simulink model "hopper_6dof"  (R2026b)
settings: Solver=FixedStepAuto  StopTime=tgrid(end)  FixedStep=1e-3  RelTol=1e-5
undefined symbols (not defined in the file): cg_init, controller_start_time, fdir_params, fsw_latency, fsw_period, g, IN, K1flat, K1flat_lo, K2grid, Klqi, nav_dt, nav_g, nav_init, nav_Qc, nav_reset, OUT, p, sensor_params, Target_Trajectory, tgrid, u_hold_command, unom, VEH
libraries: fl_lib x43, nesl_utility x31, SimscapeFluids_lib x13, slpidlib x3, simulink_extras x2, commrandsrc3 x1, dspsrcs4 x1, matrix_library x1, aerolibutil x1
(part 2 of 6)

== system hopper_6dof/Logging/Scopes_slosh/On ==
  dyn_bus : Inport
  mux : Mux  Inputs=2
  sel_dyn_bus : BusSelector  OutputSignals=ox_slosh_pos,fu_slosh_pos,ox_slosh_mass,fu_slosh_mass,f_body,cg_accel
  slosh : Scope  NumInputPorts=5
      settings: ActiveDisplayString=5  Title=CG acceleration (m/s^2)
  wires:
  mux/1 -> slosh/3
  sel_dyn_bus/5 -> slosh/4  "<f_body>"
  sel_dyn_bus/3 -> mux/1  "<ox_slosh_mass>"
  sel_dyn_bus/1 -> slosh/1  "<ox_slosh_pos>"
  dyn_bus/1 -> sel_dyn_bus/1
  sel_dyn_bus/6 -> slosh/5  "<cg_accel>"
  sel_dyn_bus/4 -> mux/2  "<fu_slosh_mass>"
  sel_dyn_bus/2 -> slosh/2  "<fu_slosh_pos>"

== system hopper_6dof/Logging/Scopes_trajectory/On ==
  dyn_bus : Inport
  mux : Mux  Inputs=2
  mux1 : Mux  Inputs=2
  mux2 : Mux  Inputs=2
  sel_dyn_bus : BusSelector  OutputSignals=x,y,z,w,vel_ned
  trajectory : Scope  NumInputPorts=4
      settings: ActiveDisplayString=4  Title=Velocity NED (m/s)  ActiveDisplayYMinimum=-1.7884841658512411  ActiveDisplayYMaximum=1.6649835435575939
  vz_ref_ts : FromWorkspace  VariableName=vz_ref_ts
  z_ref_ts : FromWorkspace  VariableName=z_ref_ts
  wires:
  sel_dyn_bus/5 -> trajectory/4  "<vel_ned>"
  sel_dyn_bus/3 -> mux1/1  "<z>"
  sel_dyn_bus/1 -> mux/1  "<x>"
  dyn_bus/1 -> sel_dyn_bus/1
  sel_dyn_bus/4 -> mux2/1  "<w>"
  sel_dyn_bus/2 -> mux/2  "<y>"
  z_ref_ts/1 -> mux1/2  "z_ref_ts"
  vz_ref_ts/1 -> mux2/2  "vz_ref_ts"
  mux/1 -> trajectory/1
  mux1/1 -> trajectory/2
  mux2/1 -> trajectory/3

== system hopper_6dof/Logging/Signal_Dump/On ==
  env_bus : Inport
  nav_bus : Inport  Port=2
  gnc_bus : Inport  Port=3
  act_bus : Inport  Port=4
  prop_bus : Inport  Port=5
  dyn_bus : Inport  Port=6
  end_act_bus : Terminator
  end_dyn_bus : Terminator
  end_env_bus : Terminator
  end_gnc_bus : Terminator
  end_nav_bus : Terminator
  end_prop_bus : Terminator
  wires:
  env_bus/1 -> end_env_bus/1
  nav_bus/1 -> end_nav_bus/1
  gnc_bus/1 -> end_gnc_bus/1
  act_bus/1 -> end_act_bus/1
  prop_bus/1 -> end_prop_bus/1
  dyn_bus/1 -> end_dyn_bus/1

== system hopper_6dof/Mass_Propulsion/Propellant_Flow/Flow_Constant ==
  Ox_mdot_in : Inport
  Fu_mdot_in : Inport  Port=2
  Unused1 : Terminator
  Unused2 : Terminator
  Zero1 : Constant  Value=0
  Zero2 : Constant  Value=0
  Ox_mdot : Outport
  Fu_mdot : Outport  Port=2
  wires:
  Ox_mdot_in/1 -> Unused1/1
  Fu_mdot_in/1 -> Unused2/1
  Zero1/1 -> Ox_mdot/1
  Zero2/1 -> Fu_mdot/1

== system hopper_6dof/Mass_Propulsion/Propellant_Flow/Flow_Varying ==
  Ox_mdot_in : Inport
  Fu_mdot_in : Inport  Port=2
  Ox_mdot : Outport
  Fu_mdot : Outport  Port=2
  wires:
  Ox_mdot_in/1 -> Ox_mdot/1
  Fu_mdot_in/1 -> Fu_mdot/1

== system hopper_6dof/Mass_Propulsion/Propulsion/Propulsion_Fluid_Network ==
  Thrust_Cmd : Inport
  Fluid_Network : Subsystem
  Thrust : Outport
  Ox_mdot : Outport  Port=2
  Fu_mdot : Outport  Port=3
  wires:
  Thrust_Cmd/1 -> Fluid_Network/1(F_cmd)
  Fluid_Network/1(Actual Thrust) -> Thrust/1  "actual_thrust_N"
  Fluid_Network/2(Actual Ox mdot) -> Ox_mdot/1  "actual_ox_mdot_kgps"
  Fluid_Network/3(Actual Fuel mdot) -> Fu_mdot/1  "actual_fuel_mdot_kgps"

== system hopper_6dof/Mass_Propulsion/Propulsion/Propulsion_LUT ==
  Thrust_Cmd : Inport
  Thrust_to_Mdot_LUT : Subsystem  ReferencedSubsystem=Thrust_to_Mdot_LUT
  Thrust : Outport
  Ox_mdot : Outport  Port=2
  Fu_mdot : Outport  Port=3
  wires:
  Thrust_Cmd/1 -> Thrust/1, Thrust_to_Mdot_LUT/1
  Thrust_to_Mdot_LUT/1 -> Ox_mdot/1
  Thrust_to_Mdot_LUT/2 -> Fu_mdot/1

== system hopper_6dof/Navigation_Sensors/FSW_Sensor_Ports/FSW_Sensor_Ports_On ==
  meas : Inport
  valid : Inport  Port=2
  stamp : Inport  Port=3
  sens_meas : Outport
  sens_valid : Outport  Port=2
  sens_stamp : Outport  Port=3
  wires:
  meas/1 -> sens_meas/1
  valid/1 -> sens_valid/1
  stamp/1 -> sens_stamp/1

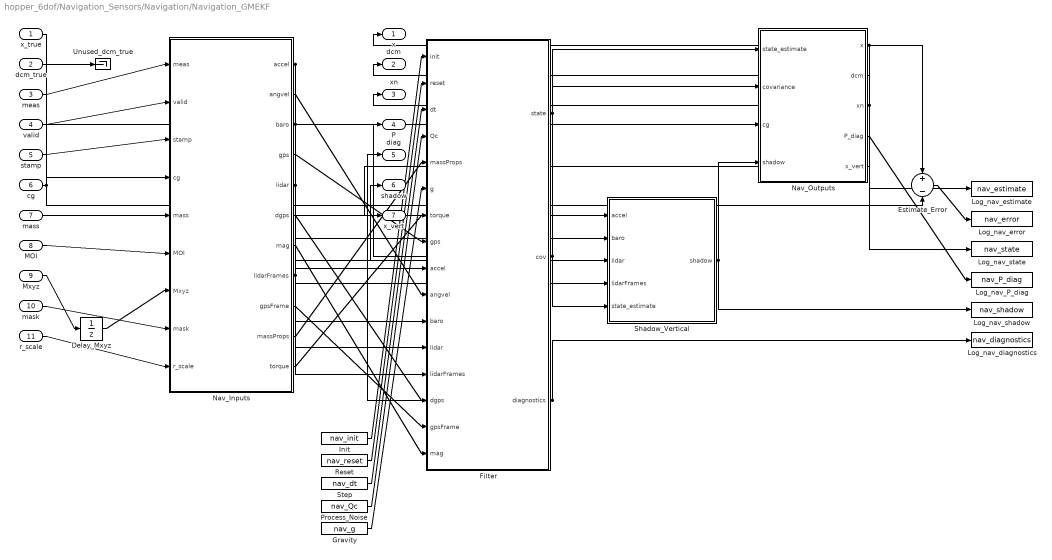
== system hopper_6dof/Navigation_Sensors/Navigation/Navigation_GMEKF ==
  x_true : Inport
  dcm_true : Inport  Port=2
  meas : Inport  Port=3
  valid : Inport  Port=4
  stamp : Inport  Port=5
  cg : Inport  Port=6
  mass : Inport  Port=7
  MOI : Inport  Port=8
  Mxyz : Inport  Port=9
  mask : Inport  Port=10
  r_scale : Inport  Port=11
  Delay_Mxyz : UnitDelay  InitialCondition=zeros(3,1)  SampleTime=nav_dt
  Estimate_Error : Sum  Inputs=+-
  Filter : Subsystem  Variant=on
  Gravity : Constant  Value=nav_g
  Init : Constant  Value=nav_init  OutDataTypeStr=Bus: InitConditions
  Log_nav_P_diag : ToWorkspace  VariableName=nav_P_diag  SaveFormat=Timeseries
  Log_nav_diagnostics : ToWorkspace  VariableName=nav_diagnostics  SaveFormat=Timeseries
  Log_nav_error : ToWorkspace  VariableName=nav_error  SaveFormat=Timeseries
  Log_nav_estimate : ToWorkspace  VariableName=nav_estimate  SaveFormat=Timeseries
  Log_nav_shadow : ToWorkspace  VariableName=nav_shadow  SaveFormat=Timeseries
  Log_nav_state : ToWorkspace  VariableName=nav_state  SaveFormat=Timeseries
  Nav_Inputs : MATLAB Function  TreatAsAtomicUnit=on  SystemSampleTime=nav_dt
  Nav_Outputs : MATLAB Function  TreatAsAtomicUnit=on
  Process_Noise : Constant  Value=nav_Qc
  Reset : Constant  Value=nav_reset
  Shadow_Vertical : MATLAB Function  TreatAsAtomicUnit=on  SystemSampleTime=nav_dt
  Step : Constant  Value=nav_dt
  Unused_dcm_true : Terminator
  x : Outport
  dcm : Outport  Port=2
  xn : Outport  Port=3
  P : Outport  Port=4
  diag : Outport  Port=5
  shadow : Outport  Port=6
  x_vert : Outport  Port=7
  wires:
  Mxyz/1 -> Delay_Mxyz/1
  meas/1 -> Nav_Inputs/1(meas)
  valid/1 -> Nav_Inputs/2(valid)
  stamp/1 -> Nav_Inputs/3(stamp)
  cg/1 -> Nav_Inputs/4(cg), Nav_Outputs/3(cg)
  mass/1 -> Nav_Inputs/5(mass)
  MOI/1 -> Nav_Inputs/6(MOI)
  Delay_Mxyz/1 -> Nav_Inputs/7(Mxyz)
  mask/1 -> Nav_Inputs/8(mask)
  r_scale/1 -> Nav_Inputs/9(r_scale)
  Init/1 -> Filter/1(init)
  Reset/1 -> Filter/2(reset)
  Step/1 -> Filter/3(dt)
  Process_Noise/1 -> Filter/4(Qc)
  Nav_Inputs/10(massProps) -> Filter/5(massProps)
  Gravity/1 -> Filter/6(g)
  Nav_Inputs/11(torque) -> Filter/7(torque)
  Nav_Inputs/4(gps) -> Filter/8(gps)
  Nav_Inputs/1(accel) -> Filter/9(accel), Shadow_Vertical/1(accel)
  Nav_Inputs/2(angvel) -> Filter/10(angvel)
  Nav_Inputs/3(baro) -> Filter/11(baro), Shadow_Vertical/2(baro)
  Nav_Inputs/5(lidar) -> Filter/12(lidar), Shadow_Vertical/3(lidar)
  Nav_Inputs/8(lidarFrames) -> Filter/13(lidarFrames), Shadow_Vertical/4(lidarFrames)
  Nav_Inputs/6(dgps) -> Filter/14(dgps)
  Nav_Inputs/9(gpsFrame) -> Filter/15(gpsFrame)
  Nav_Inputs/7(mag) -> Filter/16(mag)
  Filter/1(state) -> Shadow_Vertical/5(state_estimate), Nav_Outputs/1(state_estimate)
  Filter/2(cov) -> Nav_Outputs/2(covariance), P/1
  Shadow_Vertical/1(shadow) -> Nav_Outputs/4(shadow), shadow/1, Log_nav_shadow/1
  Nav_Outputs/3(xn) -> xn/1, Log_nav_state/1
  Filter/3(diagnostics) -> diag/1, Log_nav_diagnostics/1
  Nav_Outputs/1(x) -> Estimate_Error/1, Log_nav_estimate/1, x/1
  x_true/1 -> Estimate_Error/2
  Estimate_Error/1 -> Log_nav_error/1
  Nav_Outputs/4(P_diag) -> Log_nav_P_diag/1
  Nav_Outputs/2(dcm) -> dcm/1
  Nav_Outputs/5(x_vert) -> x_vert/1
  dcm_true/1 -> Unused_dcm_true/1

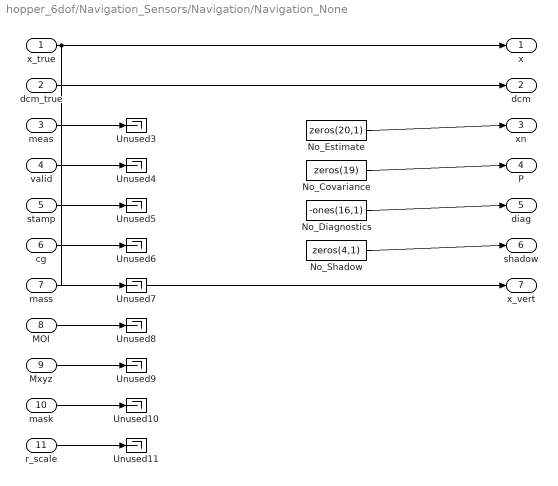
== system hopper_6dof/Navigation_Sensors/Navigation/Navigation_None ==
  x_true : Inport
  dcm_true : Inport  Port=2
  meas : Inport  Port=3
  valid : Inport  Port=4
  stamp : Inport  Port=5
  cg : Inport  Port=6
  mass : Inport  Port=7
  MOI : Inport  Port=8
  Mxyz : Inport  Port=9
  mask : Inport  Port=10
  r_scale : Inport  Port=11
  No_Covariance : Constant  Value=zeros(19)
  No_Diagnostics : Constant  Value=-ones(16,1)
  No_Estimate : Constant  Value=zeros(20,1)
  No_Shadow : Constant  Value=zeros(4,1)
  Unused{3..11} (9 alike) : Terminator
  x : Outport
  dcm : Outport  Port=2
  xn : Outport  Port=3
  P : Outport  Port=4
  diag : Outport  Port=5
  shadow : Outport  Port=6
  x_vert : Outport  Port=7
  wires:
  x_true/1 -> x/1, x_vert/1
  dcm_true/1 -> dcm/1
  No_Estimate/1 -> xn/1
  No_Covariance/1 -> P/1
  No_Diagnostics/1 -> diag/1
  No_Shadow/1 -> shadow/1
  meas/1 -> Unused3/1
  valid/1 -> Unused4/1
  stamp/1 -> Unused5/1
  cg/1 -> Unused6/1
  mass/1 -> Unused7/1
  MOI/1 -> Unused8/1
  Mxyz/1 -> Unused9/1
  mask/1 -> Unused10/1
  r_scale/1 -> Unused11/1

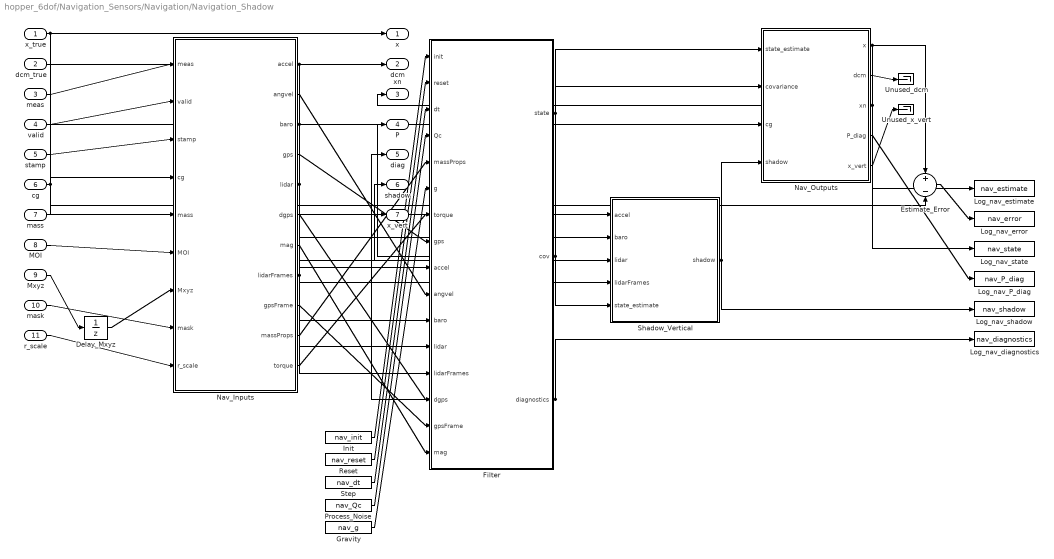
== system hopper_6dof/Navigation_Sensors/Navigation/Navigation_Shadow ==
  x_true : Inport
  dcm_true : Inport  Port=2
  meas : Inport  Port=3
  valid : Inport  Port=4
  stamp : Inport  Port=5
  cg : Inport  Port=6
  mass : Inport  Port=7
  MOI : Inport  Port=8
  Mxyz : Inport  Port=9
  mask : Inport  Port=10
  r_scale : Inport  Port=11
  Delay_Mxyz : UnitDelay  InitialCondition=zeros(3,1)  SampleTime=nav_dt
  Estimate_Error : Sum  Inputs=+-
  Filter : Subsystem  Variant=on
  Gravity : Constant  Value=nav_g
  Init : Constant  Value=nav_init  OutDataTypeStr=Bus: InitConditions
  Log_nav_P_diag : ToWorkspace  VariableName=nav_P_diag  SaveFormat=Timeseries
  Log_nav_diagnostics : ToWorkspace  VariableName=nav_diagnostics  SaveFormat=Timeseries
  Log_nav_error : ToWorkspace  VariableName=nav_error  SaveFormat=Timeseries
  Log_nav_estimate : ToWorkspace  VariableName=nav_estimate  SaveFormat=Timeseries
  Log_nav_shadow : ToWorkspace  VariableName=nav_shadow  SaveFormat=Timeseries
  Log_nav_state : ToWorkspace  VariableName=nav_state  SaveFormat=Timeseries
  Nav_Inputs : MATLAB Function  TreatAsAtomicUnit=on  SystemSampleTime=nav_dt
  Nav_Outputs : MATLAB Function  TreatAsAtomicUnit=on
  Process_Noise : Constant  Value=nav_Qc
  Reset : Constant  Value=nav_reset
  Shadow_Vertical : MATLAB Function  TreatAsAtomicUnit=on  SystemSampleTime=nav_dt
  Step : Constant  Value=nav_dt
  Unused_dcm : Terminator
  Unused_x_vert : Terminator
  x : Outport
  dcm : Outport  Port=2
  xn : Outport  Port=3
  P : Outport  Port=4
  diag : Outport  Port=5
  shadow : Outport  Port=6
  x_vert : Outport  Port=7
  wires:
  Mxyz/1 -> Delay_Mxyz/1
  meas/1 -> Nav_Inputs/1(meas)
  valid/1 -> Nav_Inputs/2(valid)
  stamp/1 -> Nav_Inputs/3(stamp)
  cg/1 -> Nav_Inputs/4(cg), Nav_Outputs/3(cg)
  mass/1 -> Nav_Inputs/5(mass)
  MOI/1 -> Nav_Inputs/6(MOI)
  Delay_Mxyz/1 -> Nav_Inputs/7(Mxyz)
  mask/1 -> Nav_Inputs/8(mask)
  r_scale/1 -> Nav_Inputs/9(r_scale)
  Init/1 -> Filter/1(init)
  Reset/1 -> Filter/2(reset)
  Step/1 -> Filter/3(dt)
  Process_Noise/1 -> Filter/4(Qc)
  Nav_Inputs/10(massProps) -> Filter/5(massProps)
  Gravity/1 -> Filter/6(g)
  Nav_Inputs/11(torque) -> Filter/7(torque)
  Nav_Inputs/4(gps) -> Filter/8(gps)
  Nav_Inputs/1(accel) -> Filter/9(accel), Shadow_Vertical/1(accel)
  Nav_Inputs/2(angvel) -> Filter/10(angvel)
  Nav_Inputs/3(baro) -> Filter/11(baro), Shadow_Vertical/2(baro)
  Nav_Inputs/5(lidar) -> Filter/12(lidar), Shadow_Vertical/3(lidar)
  Nav_Inputs/8(lidarFrames) -> Filter/13(lidarFrames), Shadow_Vertical/4(lidarFrames)
  Nav_Inputs/6(dgps) -> Filter/14(dgps)
  Nav_Inputs/9(gpsFrame) -> Filter/15(gpsFrame)
  Nav_Inputs/7(mag) -> Filter/16(mag)
  Filter/1(state) -> Shadow_Vertical/5(state_estimate), Nav_Outputs/1(state_estimate)
  Filter/2(cov) -> Nav_Outputs/2(covariance), P/1
  Shadow_Vertical/1(shadow) -> Nav_Outputs/4(shadow), shadow/1, Log_nav_shadow/1
  Nav_Outputs/3(xn) -> xn/1, Log_nav_state/1
  Filter/3(diagnostics) -> diag/1, Log_nav_diagnostics/1
  Nav_Outputs/1(x) -> Estimate_Error/1, Log_nav_estimate/1
  x_true/1 -> Estimate_Error/2, x/1, x_vert/1
  Estimate_Error/1 -> Log_nav_error/1
  Nav_Outputs/4(P_diag) -> Log_nav_P_diag/1
  dcm_true/1 -> dcm/1
  Nav_Outputs/2(dcm) -> Unused_dcm/1
  Nav_Outputs/5(x_vert) -> Unused_x_vert/1

== system hopper_6dof/Navigation_Sensors/Sensors/Sensors_Off ==
  x : Inport
  f_b : Inport  Port=2
  dcm_be : Inport  Port=3
  cg : Inport  Port=4
  Unused{1..4} (4 alike) : Terminator
  Zero1 : Constant  Value=zeros(26,1)
  Zero2 : Constant  Value=zeros(9,1)
  Zero3 : Constant  Value=zeros(9,1)
  meas : Outport
  valid : Outport  Port=2
  stamp : Outport  Port=3
  wires:
  x/1 -> Unused1/1
  f_b/1 -> Unused2/1
  dcm_be/1 -> Unused3/1
  cg/1 -> Unused4/1
  Zero1/1 -> meas/1
  Zero2/1 -> valid/1
  Zero3/1 -> stamp/1

== system hopper_6dof/Navigation_Sensors/Sensors/Sensors_On ==
  x : Inport
  f_b : Inport  Port=2
  dcm_be : Inport  Port=3
  cg : Inport  Port=4
  Clock : Clock
  Sensor_Frame : MATLAB Function  TreatAsAtomicUnit=on  SystemSampleTime=sensor_params.dt
  Sensor_Noise : RandomNumber  Mean=zeros(26,1)  Variance=ones(26,1)  Seed=sensor_params.S.seed + (0:25)'  SampleTime=sensor_params.dt
  meas : Outport
  valid : Outport  Port=2
  stamp : Outport  Port=3
  wires:
  Clock/1 -> Sensor_Frame/1(t)
  Sensor_Noise/1 -> Sensor_Frame/2(noise)
  x/1 -> Sensor_Frame/3(x)
  f_b/1 -> Sensor_Frame/4(f_b)
  dcm_be/1 -> Sensor_Frame/5(dcm_be)
  cg/1 -> Sensor_Frame/6(cg)
  Sensor_Frame/1(meas) -> meas/1
  Sensor_Frame/2(valid) -> valid/1
  Sensor_Frame/3(stamp) -> stamp/1

== system hopper_6dof/Vehicle_Dynamics/Ground_Contact/Ground_None ==
  Inertial Position : Inport
  Inertial Velocity : Inport  Port=2
  Inertial to Body : Inport  Port=3
  Angular Velocity : Inport  Port=4
  Unused{1..4} (4 alike) : Terminator
  Zero1 : Constant  Value=[0 0 0]
  Zero2 : Constant  Value=[0 0 0]
  Body Force : Outport
  Body Moment : Outport  Port=2
  wires:
  Inertial Position/1 -> Unused1/1
  Inertial Velocity/1 -> Unused2/1
  Inertial to Body/1 -> Unused3/1
  Angular Velocity/1 -> Unused4/1
  Zero1/1 -> Body Force/1
  Zero2/1 -> Body Moment/1

== system hopper_6dof/Vehicle_Dynamics/Ground_Contact/Ground_Strut ==
  Inertial Position : Inport
  Inertial Velocity : Inport  Port=2
  Inertial to Body : Inport  Port=3
  Angular Velocity : Inport  Port=4
  Ground_Contact : Subsystem  ReferencedSubsystem=Ground_Contact
  Body Force : Outport
  Body Moment : Outport  Port=2
  wires:
  Inertial Position/1 -> Ground_Contact/1
  Inertial Velocity/1 -> Ground_Contact/2
  Inertial to Body/1 -> Ground_Contact/3
  Angular Velocity/1 -> Ground_Contact/4
  Ground_Contact/1 -> Body Force/1
  Ground_Contact/2 -> Body Moment/1

== system hopper_6dof/Vehicle_Dynamics/Slosh/Slosh_Off ==
  Ox mass : Inport
  Fuel mass : Inport  Port=2
  CG Acceleration : Inport  Port=3
  Angular Velocity : Inport  Port=4
  Angular Acceleration : Inport  Port=5
  CG Location : Inport  Port=6
  Unused{1..6} (6 alike) : Terminator
  Zero{1,3..6} (5 alike) : Constant  Value=[0 0 0]
  Zero2 : Constant  Value=zeros(3,1)
  Slosh_F : Outport
  Slosh_M : Outport  Port=2
  ox_slosh_pos : Outport  Port=3
  ox_slosh_mass : Outport  Port=4
  fu_slosh_pos : Outport  Port=5
  fu_slosh_mass : Outport  Port=6
  wires:
  Ox mass/1 -> Unused1/1
  Fuel mass/1 -> Unused2/1
  CG Acceleration/1 -> Unused3/1
  Angular Velocity/1 -> Unused4/1
  Angular Acceleration/1 -> Unused5/1
  CG Location/1 -> Unused6/1
  Zero1/1 -> Slosh_F/1
  Zero2/1 -> Slosh_M/1
  Zero3/1 -> ox_slosh_pos/1
  Zero4/1 -> ox_slosh_mass/1
  Zero5/1 -> fu_slosh_pos/1
  Zero6/1 -> fu_slosh_mass/1

== system hopper_6dof/GNC/Controller/Controller_LQI/MRP Correction ==
  In1 : Inport
  Constant : Constant  Value=p(2)
  Demux : Demux  Outputs=3
  Mux : Mux  Inputs=3
  Sum : Sum  Inputs=|+-
  Out1 : Outport
  wires:
  Demux/1 -> Mux/1
  Demux/3 -> Mux/3
  Constant/1 -> Sum/2
  Mux/1 -> Out1/1
  Sum/1 -> Mux/2
  Demux/2 -> Sum/1
  In1/1 -> Demux/1

== system hopper_6dof/GNC/Controller/Controller_LQI/q to MRP ==
  In1 : Inport
  Constant : Constant
  Matrix Divide : Product  Inputs=*/
  Selector : Selector  InputPortWidth=4  IndexOptions=Index vector (dialog)  Indices=[1 2 3]  OutputSizes=1  RuntimeRangeChecks=off
  Selector1 : Selector  InputPortWidth=4  IndexOptions=Index vector (dialog)  Indices=[1]  OutputSizes=1  RuntimeRangeChecks=off
  Sum : Sum  Inputs=|++
  Out1 : Outport
  wires:
  Matrix Divide/1 -> Out1/1
  Sum/1 -> Matrix Divide/2
  Selector/1 -> Matrix Divide/1
  Constant/1 -> Sum/2
  Selector1/1 -> Sum/1
  In1/1 -> Selector/1, Selector1/1

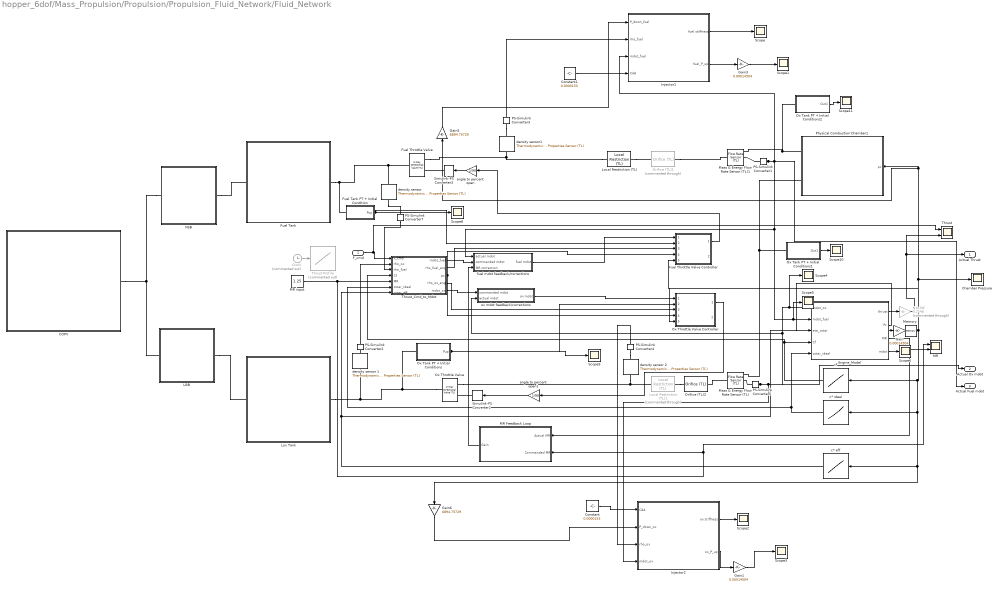
== system hopper_6dof/Mass_Propulsion/Propulsion/Propulsion_Fluid_Network/Fluid_Network ==
  F_cmd : Inport
  COPV : Subsystem
  Chamber Pressure : Scope
      settings: ActiveDisplayYMinimum=24.4768520913143  ActiveDisplayYMaximum=276.14956071215624  DataLoggingVariableName=ScopeData22
  Clock : Clock  Commented=on
  Constant : Constant  Value=0.0000153
  Constant1 : Constant  Value=0.0000153
  Engine_Model : MATLAB Function  TreatAsAtomicUnit=on
  FBB : Subsystem
  Fuel Tank : Subsystem
  Fuel Tank PT + Initial Condition : Subsystem
  Fuel Throttle Valve : SimscapeFluids_lib/Thermal Liquid/Valves & Orifices/Directional Control Valves/2-Way Directional Valve (TL)  valve_spec=fluids.thermal_liquid.valves.directional_control_valves.enum.ValveSpec.Table1DAreaOpening  S_max=1 m  del_S_max=5e-3 m  area_max=1e-4 m^2  area_leak=1e-10 m^2  del_S_TLU=[0 0.3 0.4 0.5 0.6 0.7 0.8 0.9 1.0] m  valve_area_TLU=[1e-9 1.7065e-07 1.0239e-06 3.5836e-06 7.8498e-06 1.4164e-05 2.3038e-05 3.4812e-05 5.0000e-05] m^2  del_S_flow_TLU=[0, .002, .004, .007, .017] m  p_diff_TLU=[.3, .5, .7] MPa  vol_flow_TLU=1e-3 * [1.7e-05, 2e-05, 2.6e-05; .0035, .0045, .0053; .7, .9, 1.06; 1.96, 2.5, 3; 6, 7.7, 9.13] m^3/s  mdot_TLU=[1.7e-05, 2e-05, 2.6e-05; .0035, .0045, .0053; .7, .9, 1.06; 1.96, 2.5, 3; 6, 7.7, 9.13] kg/s  T_ref_in=293.15 K  p_ref_in=0.101325 MPa  Cd=1  Re_c=150  smoothing_factor=0.01  pressure_recovery=false  area=0.01 m^2
  Fuel Throttle Valve Controller : Subsystem  ReferencedSubsystem=Throttle_Valve_Controller  ramp_slope=60
  Gain : Gain  Gain=0.00014504
  Gain1 : Gain  Gain=0.00014504
  Gain3 : Gain  Gain=0.00014504
  Gain5 : Gain  Gain=6894.75729
  Gain6 : Gain  Gain=6894.75729
  Injector1 : Subsystem
  Injector2 : Subsystem
  LBB : Subsystem
  Local Restriction (TL) : fl_lib/Thermal Liquid/Elements/Local Restriction (TL)  restriction_type=foundation.enum.restriction_type.fixed  restriction_area=0.0000153 m^2  min_area=1e-10 m^2  max_area=0.005 m^2  area=0.000153 m^2  Cd=1  Re_c=150  pressure_recovery=true
  Local Restriction (TL)1 : fl_lib/Thermal Liquid/Elements/Local Restriction (TL)  Commented=through  restriction_type=foundation.enum.restriction_type.fixed  restriction_area=0.0000153 m^2  min_area=1e-10 m^2  max_area=0.005 m^2  area=0.000153 m^2  Cd=1  Re_c=150  pressure_recovery=true
  Lox Tank : Subsystem
  MR : Scope  NumInputPorts=2
      settings: ActiveDisplayYMinimum=0.081947452963374467  ActiveDisplayYMaximum=2.5817499803566988
  MR Feedback Loop : Subsystem
  MR input : Constant  Value=1.25
  Mass & Energy Flow Rate Sensor (TL) : fl_lib/Thermal Liquid/Sensors/Flow Rate Sensor (TL)  mass_flow_measure=true  volumetric_flow_measure=false  energy_flow_measure=true
  Mass & Energy Flow Rate Sensor (TL)1 : fl_lib/Thermal Liquid/Sensors/Flow Rate Sensor (TL)  mass_flow_measure=true  volumetric_flow_measure=false  energy_flow_measure=true
  Memory : Memory  InitialCondition=300
  N to lbf : Gain  Commented=through  Gain=0.2248
  Orifice (TL)1 : SimscapeFluids_lib/Thermal Liquid/Valves & Orifices/Orifice (TL)  Commented=through  orifice_type=foundation.enum.constant_variable.constant  constant_orifice_spec=fluids.thermal_liquid.valves.enum.ConstantOrificeSpec.Area  variable_orifice_spec=fluids.thermal_liquid.valves.enum.orifice_spec.linear  orifice_area_constant=0.0000153 m^2  p_diff_TLU_constant=[-4, -3, -2, -1, -.5, 0, .5, 1, 2, 3, 4] MPa  vol_flow_TLU_constant=[-2.44, -2.12, -1.68, -1.22, -.84, 0, .85, 1.21, 1.7, 2.09, 2.41] .* 1e-3 m^3/s  mdot_TLU_constant=[-2.44, -2.12, -1.68, -1.22, -.84, 0, .85, 1.21, 1.7, 2.09, 2.41] kg/s  S_min=0 m  del_S=5e-3 m  open_orientation=fluids.thermal_liquid.valves.enum.orifice_orientation.positive  area_max=1e-4 m^2  area_leak=1e-10 m^2  S_TLU=[0, .002, .004, .007, .017] m  orifice_area_TLU=[1e-09, 2.0352e-07, 4.0736e-05, .00011438, .00034356] m^2  Cd=1  Re_c=150  smoothing_factor=0.01  pressure_recovery=false  S_flow_TLU=[0, .002, .004, .007, .017] m  p_diff_TLU=[.3, .5, .7] MPa  vol_flow_TLU=1e-3 * [1.7e-05, 2e-05, 2.6e-05; .0035, .0045, .0053; .7, .9, 1.06; 1.96, 2.5, 3; 6, 7.7, 9.13] m^3/s  mdot_TLU=[1.7e-05, 2e-05, 2.6e-05; .0035, .0045, .0053; .7, .9, 1.06; 1.96, 2.5, 3; 6, 7.7, 9.13] kg/s  T_ref_in=293.15 K  p_ref_in=0.101325 MPa  area=0.01 m^2
  Orifice (TL)2 : SimscapeFluids_lib/Thermal Liquid/Valves & Orifices/Orifice (TL)  orifice_type=foundation.enum.constant_variable.constant  constant_orifice_spec=fluids.thermal_liquid.valves.enum.ConstantOrificeSpec.Area  variable_orifice_spec=fluids.thermal_liquid.valves.enum.orifice_spec.linear  orifice_area_constant=0.0000153 m^2  p_diff_TLU_constant=[-4, -3, -2, -1, -.5, 0, .5, 1, 2, 3, 4] MPa  vol_flow_TLU_constant=[-2.44, -2.12, -1.68, -1.22, -.84, 0, .85, 1.21, 1.7, 2.09, 2.41] .* 1e-3 m^3/s  mdot_TLU_constant=[-2.44, -2.12, -1.68, -1.22, -.84, 0, .85, 1.21, 1.7, 2.09, 2.41] kg/s  S_min=0 m  del_S=5e-3 m  open_orientation=fluids.thermal_liquid.valves.enum.orifice_orientation.positive  area_max=1e-4 m^2  area_leak=1e-10 m^2  S_TLU=[0, .002, .004, .007, .017] m  orifice_area_TLU=[1e-09, 2.0352e-07, 4.0736e-05, .00011438, .00034356] m^2  Cd=1  Re_c=150  smoothing_factor=0.01  pressure_recovery=false  S_flow_TLU=[0, .002, .004, .007, .017] m  p_diff_TLU=[.3, .5, .7] MPa  vol_flow_TLU=1e-3 * [1.7e-05, 2e-05, 2.6e-05; .0035, .0045, .0053; .7, .9, 1.06; 1.96, 2.5, 3; 6, 7.7, 9.13] m^3/s  mdot_TLU=[1.7e-05, 2e-05, 2.6e-05; .0035, .0045, .0053; .7, .9, 1.06; 1.96, 2.5, 3; 6, 7.7, 9.13] kg/s  T_ref_in=293.15 K  p_ref_in=0.101325 MPa  area=0.01 m^2
  Ox Tank PT + Initial Conditions : Subsystem
  Ox Tank PT + Initial Conditions1 : Subsystem
  Ox Tank PT + Initial Conditions2 : Subsystem
  Ox Throttle Valve : SimscapeFluids_lib/Thermal Liquid/Valves & Orifices/Directional Control Valves/2-Way Directional Valve (TL)  valve_spec=fluids.thermal_liquid.valves.directional_control_valves.enum.ValveSpec.Table1DAreaOpening  S_max=1 m  del_S_max=5e-3 m  area_max=1e-4 m^2  area_leak=1e-10 m^2  del_S_TLU=[0 0.3 0.4 0.5 0.6 0.7 0.8 0.9 1.0] m  valve_area_TLU=[1e-9 1.7065e-07 1.0239e-06 3.5836e-06 7.8498e-06 1.4164e-05 2.3038e-05 3.4812e-05 5.0000e-05] m^2  del_S_flow_TLU=[0, .002, .004, .007, .017] m  p_diff_TLU=[.3, .5, .7] MPa  vol_flow_TLU=1e-3 * [1.7e-05, 2e-05, 2.6e-05; .0035, .0045, .0053; .7, .9, 1.06; 1.96, 2.5, 3; 6, 7.7, 9.13] m^3/s  mdot_TLU=[1.7e-05, 2e-05, 2.6e-05; .0035, .0045, .0053; .7, .9, 1.06; 1.96, 2.5, 3; 6, 7.7, 9.13] kg/s  T_ref_in=293.15 K  p_ref_in=0.101325 MPa  Cd=1  Re_c=150  smoothing_factor=0.01  pressure_recovery=false  area=0.01 m^2
  Ox Throttle Valve Controller : Subsystem  ReferencedSubsystem=Throttle_Valve_Controller  ramp_slope=48
  PS-Simulink Converter{1..5,7} (6 alike) : nesl_utility/PS-Simulink Converter  PhysicalDomain=network_engine_domain  SubClassName=ps_output  LeftPortType=input  RightPortType=output  PseudoPeriodic=off  Frequencies=[]  VectorFormat=inherit  Unit=inherit  AffineConversion=off
  Physical Combustion Chamber1 : Subsystem
  Scope{,1..6,8..11} (11 alike) : Scope
      Scope settings: ActiveDisplayYMinimum=-0.024254245068718681  ActiveDisplayYMaximum=0.21828827495285463  DataLoggingVariableName=ScopeData40
      Scope1 settings: ActiveDisplayYMinimum=-37.465424615708343  ActiveDisplayYMaximum=337.50135970832162  DataLoggingVariableName=ScopeData42
      Scope10 settings: ActiveDisplayYMinimum=-62.731329785992315  ActiveDisplayYMaximum=586.85713455527571  DataLoggingVariableName=ScopeData51
      Scope11 settings: ActiveDisplayYMinimum=-62.499971643181283  ActiveDisplayYMaximum=562.49999684924239  DataLoggingVariableName=ScopeData52
      Scope2 settings: ActiveDisplayYMinimum=-0.025857157768165939  ActiveDisplayYMaximum=0.4462125176132366  DataLoggingVariableName=ScopeData43
      Scope3 settings: ActiveDisplayYMinimum=-1  ActiveDisplayYMaximum=1  DataLoggingVariableName=ScopeData44
      Scope4 settings: ActiveDisplayYMinimum=-0.071595374751251564  ActiveDisplayYMaximum=0.64519605918641931  DataLoggingVariableName=ScopeData53
      Scope5 settings: ActiveDisplayYMinimum=-0.05515719954820638  ActiveDisplayYMaximum=0.49713967255882957  DataLoggingVariableName=ScopeData54
      Scope6 settings: ActiveDisplayYMinimum=-0.1205205125313115  ActiveDisplayYMaximum=1.086247175831931  DataLoggingVariableName=ScopeData55
      Scope8 settings: ActiveDisplayYMinimum=481.05362935967628  ActiveDisplayYMaximum=536.06057249536832  DataLoggingVariableName=ScopeData49
      Scope9 settings: ActiveDisplayYMinimum=492.10107740407369  ActiveDisplayYMaximum=524.51908611925091  DataLoggingVariableName=ScopeData50
  Simulink-PS Converter2 : nesl_utility/Simulink-PS Converter  PhysicalDomain=network_engine_domain  SubClassName=ps_input  LeftPortType=input  RightPortType=output  PseudoPeriodic=off  Frequencies=[]  NoiseDistribution=none  NoiseParameters=[]  Unit=1  AffineConversion=off  FilteringAndDerivatives=filter  SimscapeFilterOrder=1  InputFilterTimeConstant=0.001  UdotUserProvided=0
  Simulink-PS Converter3 : nesl_utility/Simulink-PS Converter  PhysicalDomain=network_engine_domain  SubClassName=ps_input  LeftPortType=input  RightPortType=output  PseudoPeriodic=off  Frequencies=[]  NoiseDistribution=none  NoiseParameters=[]  Unit=1  AffineConversion=off  FilteringAndDerivatives=filter  SimscapeFilterOrder=1  InputFilterTimeConstant=0.001  UdotUserProvided=0
  Thrust : Scope  NumInputPorts=2
      settings: ActiveDisplayYMinimum=-215.53569406218494  ActiveDisplayYMaximum=1942.1553478833205  DataLoggingVariableName=ScopeData21
  Thrust Profile : Lookup_n-D  Commented=on  NumberOfTableDimensions=1  BreakpointsForDimension1=|  Table=|  InternalRulePriority=Speed  RndMeth=Simplest
      BreakpointsForDimension1=|
      | [0
      | 2.46e-15
      | 4.93e-15
      | 1.31e-14
      | 1.85798e-4
      | 3.71595e-4
      | 1.300583e-3
      | 5.945524e-3
      | 2.917023e-2
      | 1.452937e-1
      | 3.251823e-1
      | 6.176896e-1
      | 1.048884
      | 1.648122
      | 2.452841
      | 3.452841
      | 4.452841
      | 5.452841
      | 6.452841
      | 7.452841
      | 8.452841
      | 9.452841
      | 10.45284
      | 11.45284
      | 12.45284
      | 13.45284
      | 14.45284
      | 15.45284
      | 16.26888
      | 17.26888
      | 18.26888
      | 19.26888
      | 20.26888
      | 21.26888
      | 21.82014
      | 22.37140
      | 23.10183
      | 24.10183
      | 25.10183
      | 26.10183
      | 27.10183
      | 28.10183
      | 29.10183
      | 29.70287]
      Table=|
      | [1115.929794
      | 1115.929794
      | 1115.929794
      | 1115.929794
      | 1116.015031
      | 1116.100248
      | 1116.526042
      | 1118.647732
      | 1129.075722
      | 1176.888468
      | 1237.984070
      | 1309.087819
      | 1365.657208
      | 1382.500173
      | 1347.869214
      | 1276.732855
      | 1209.886660
      | 1007.359221
      | 890.000000
      | 890.000000
      | 890.000000
      | 890.000000
      | 970.372958
      | 1015.368113
      | 1034.720854
      | 1040.888013
      | 1040.596927
      | 896.870767
      | 890.000000
      | 890.000000
      | 890.000000
      | 890.000000
      | 890.000000
      | 890.000000
      | 1074.062231
      | 1213.486737
      | 1218.338865
      | 1172.384789
      | 1114.978943
      | 1066.195681
      | 1030.043331
      | 1004.841448
      | 987.599936
      | 979.912878]
  Thrust_Cmd_to_Mdot : MATLAB Function  TreatAsAtomicUnit=on
  angle to percent open : Gain  Gain=1/90
  angle to percent open1 : Gain  Gain=1/90
  c* eff : Lookup_n-D  NumberOfTableDimensions=1  BreakpointsForDimension1=[125 295]  Table=[0.8 0.85]  InternalRulePriority=Speed  RndMeth=Simplest
  c* ideal : Lookup_n-D  NumberOfTableDimensions=1  BreakpointsForDimension1=[100 110 120 130 140 150 160 170 180 190 200 210 220 230 240 250 260 270 280 290 300 310 320 330 340 350]  Table=[1492.810749 1492.812678 1492.815823 1492.820080 1492.825344 1492.831574 1492.838703 1492.846662 1492.855462 1492.865052 1492.875406 1492.886504 1492.898325 1492.910854 1492.924078 1492.937982 1492.952558 1492.967791 1492.983688 1493.000184 1493.017345 1493.035113 1493.053494 1493.072480 1493.092063 1493.112237]  InternalRulePriority=Speed  RndMeth=Simplest
  cf : Lookup_n-D  NumberOfTableDimensions=1  BreakpointsForDimension1=[125 295]  Table=[1.42 1.57]  InternalRulePriority=Speed  RndMeth=Simplest
  density sensor : fl_lib/Thermal Liquid/Sensors/Thermodynamic Properties Sensor (TL)  internal_energy=false  density=true  specific_heat=false
  density sensor 1 : fl_lib/Thermal Liquid/Sensors/Thermodynamic Properties Sensor (TL)  internal_energy=false  density=true  specific_heat=false
  density sensor 2 : fl_lib/Thermal Liquid/Sensors/Thermodynamic Properties Sensor (TL)  internal_energy=false  density=true  specific_heat=false
  density sensor1 : fl_lib/Thermal Liquid/Sensors/Thermodynamic Properties Sensor (TL)  internal_energy=false  density=true  specific_heat=false
  fuel mdot feedback/corrections : Subsystem
  ox mdot feedback/corrections : Subsystem
  Actual Thrust : Outport
  Actual Ox mdot : Outport  Port=2
  Actual Fuel mdot : Outport  Port=3
  wires:
  Ox Throttle Valve Controller/1 -> angle to percent open1/1
  Thrust_Cmd_to_Mdot/4(rho_ox_eng) -> Ox Throttle Valve Controller/3
  ox mdot feedback/corrections/1(ox mdot) -> Ox Throttle Valve Controller/1
  Fuel Throttle Valve Controller/1 -> angle to percent open/1
  Thrust_Cmd_to_Mdot/2(rho_fuel_eng) -> Fuel Throttle Valve Controller/3
  fuel mdot feedback/corrections/1(fuel mdot) -> Fuel Throttle Valve Controller/1
  Engine_Model/4(mdot) -> Scope6/1
  PS-Simulink Converter4/1 -> Injector2/3(rho_ox)
  PS-Simulink Converter3/1 -> Injector1/2(rho_fuel)
  Memory/1 -> Ox Throttle Valve Controller/5, Fuel Throttle Valve Controller/5, Chamber Pressure/1, Physical Combustion Chamber1/1(pc), Gain5/1, cf/1, c* ideal/1, c* eff/1, Gain6/1
  Gain6/1 -> Injector2/2(P_down_ox)
  Gain5/1 -> Injector1/1(P_down_fuel)
  Gain1/1 -> Scope3/1
  Gain3/1 -> Scope1/1
  Ox Tank PT + Initial Conditions2/1(Out1) -> Scope11/1
  Ox Tank PT + Initial Conditions1/1(Out1) -> Scope10/1
  PS-Simulink Converter7/1 -> Thrust_Cmd_to_Mdot/3(rho_fuel)
  Constant1/1 -> Injector1/4(CdA)
  Constant/1 -> Injector2/1(CdA)
  Injector2/2(ox_P_up) -> Gain1/1
  Injector2/1(ox stiffness) -> Scope2/1
  Injector1/2(fuel_P_up) -> Gain3/1
  Injector1/1(fuel stiffness) -> Scope/1
  PS-Simulink Converter1/1 -> fuel mdot feedback/corrections/1(actual mdot), Engine_Model/2(mdot_fuel), Scope5/1, Injector1/3(mdot_fuel), Actual Fuel mdot/1
  PS-Simulink Converter5/1 -> ox mdot feedback/corrections/2(actual mdot), Engine_Model/1(mdot_ox), Scope4/1, Injector2/4(mdot_ox), Actual Ox mdot/1
  F_cmd/1 -> Thrust_Cmd_to_Mdot/1(F_cmd), Thrust/1
  cf/1 -> Engine_Model/4(Cf), Thrust_Cmd_to_Mdot/4(Cf)
  c* eff/1 -> Engine_Model/3(eta_cstar), Thrust_Cmd_to_Mdot/7(cstar_eff)
  PS-Simulink Converter2/1 -> Thrust_Cmd_to_Mdot/2(rho_ox)
  Thrust_Cmd_to_Mdot/3(pc) -> Ox Throttle Valve Controller/4, Fuel Throttle Valve Controller/4
  MR input/1 -> Thrust_Cmd_to_Mdot/5(MR), MR/1, MR Feedback Loop/2(Commanded MR)
  MR Feedback Loop/1(Gain) -> fuel mdot feedback/corrections/3(MR correction)
  Engine_Model/2(Pc) -> Gain/1
  Gain/1 -> Memory/1
  Engine_Model/1(thrust) -> N to lbf/1
  Clock/1 -> Thrust Profile/1
  Thrust_Cmd_to_Mdot/5(mdot_ox) -> ox mdot feedback/corrections/1(commanded mdot)
  Engine_Model/3(MR) -> MR/2, MR Feedback Loop/1(Actual MR)
  angle to percent open1/1 -> Simulink-PS Converter2/1
  angle to percent open/1 -> Simulink-PS Converter3/1
  Ox Tank PT + Initial Conditions/1(Pup) -> Ox Throttle Valve Controller/2, Scope9/1
  Thrust_Cmd_to_Mdot/1(mdot_fuel) -> fuel mdot feedback/corrections/2(commanded mdot)
  N to lbf/1 -> Actual Thrust/1, Thrust/2
  Fuel Tank PT + Initial Condition/1(Pup) -> Fuel Throttle Valve Controller/2, Scope8/1
  c* ideal/1 -> Thrust_Cmd_to_Mdot/6(cstar_ideal), Engine_Model/5(cstar_ideal)
  connections:
  Local Restriction (TL)1/RConn1 -- Orifice (TL)2/LConn1
  Local Restriction (TL)/RConn1 -- Orifice (TL)1/LConn1
  PS-Simulink Converter4/LConn1 -- density sensor 2/RConn1
  PS-Simulink Converter3/LConn1 -- density sensor1/RConn1
  Orifice (TL)2/RConn1 -- Mass & Energy Flow Rate Sensor (TL)/LConn1
  Orifice (TL)1/RConn1 -- Mass & Energy Flow Rate Sensor (TL)1/LConn1
  Local Restriction (TL)/LConn1 -- density sensor1/LConn1 -- Fuel Throttle Valve/RConn2
  Simulink-PS Converter2/RConn1 -- Ox Throttle Valve/RConn1
  PS-Simulink Converter1/LConn1 -- Mass & Energy Flow Rate Sensor (TL)1/RConn2
  FBB/LConn1 -- LBB/LConn1 -- COPV/RConn1
  Ox Throttle Valve/LConn1 -- Ox Tank PT + Initial Conditions/LConn1 -- density sensor 1/LConn1 -- Lox Tank/RConn1
  density sensor/RConn1 -- PS-Simulink Converter7/LConn1
  Mass & Energy Flow Rate Sensor (TL)/RConn1 -- Physical Combustion Chamber1/RConn2 -- Ox Tank PT + Initial Conditions1/LConn1
  FBB/RConn1 -- Fuel Tank/LConn1
  Ox Tank PT + Initial Conditions2/LConn1 -- Physical Combustion Chamber1/RConn1 -- Mass & Energy Flow Rate Sensor (TL)1/RConn1
  density sensor 2/LConn1 -- Local Restriction (TL)1/LConn1 -- Ox Throttle Valve/RConn2
  PS-Simulink Converter5/LConn1 -- Mass & Energy Flow Rate Sensor (TL)/RConn2
  Simulink-PS Converter3/RConn1 -- Fuel Throttle Valve/RConn1
  Fuel Tank PT + Initial Condition/LConn1 -- Fuel Tank/RConn1 -- density sensor/LConn1 -- Fuel Throttle Valve/LConn1
  LBB/RConn1 -- Lox Tank/LConn1
  density sensor 1/RConn1 -- PS-Simulink Converter2/LConn1

== system hopper_6dof/Navigation_Sensors/Navigation/Navigation_GMEKF/Filter ==
  init : Inport
  reset : Inport  Port=2
  dt : Inport  Port=3
  Qc : Inport  Port=4
  massProps : Inport  Port=5
  g : Inport  Port=6
  torque : Inport  Port=7
  gps : Inport  Port=8
  accel : Inport  Port=9
  angvel : Inport  Port=10
  baro : Inport  Port=11
  lidar : Inport  Port=12
  lidarFrames : Inport  Port=13
  dgps : Inport  Port=14
  gpsFrame : Inport  Port=15
  mag : Inport  Port=16
  Filter_CTV : Subsystem  VariantControl=VARIANT_VEHICLE == 2
  Filter_Hopper : Subsystem  VariantControl=VARIANT_VEHICLE == 1
  state : Outport
  cov : Outport  Port=2
  diagnostics : Outport  Port=3

== system hopper_6dof/Navigation_Sensors/Navigation/Navigation_Shadow/Filter ==
  init : Inport
  reset : Inport  Port=2
  dt : Inport  Port=3
  Qc : Inport  Port=4
  massProps : Inport  Port=5
  g : Inport  Port=6
  torque : Inport  Port=7
  gps : Inport  Port=8
  accel : Inport  Port=9
  angvel : Inport  Port=10
  baro : Inport  Port=11
  lidar : Inport  Port=12
  lidarFrames : Inport  Port=13
  dgps : Inport  Port=14
  gpsFrame : Inport  Port=15
  mag : Inport  Port=16
  Filter_CTV : Subsystem  VariantControl=VARIANT_VEHICLE == 2
  Filter_Hopper : Subsystem  VariantControl=VARIANT_VEHICLE == 1
  state : Outport
  cov : Outport  Port=2
  diagnostics : Outport  Port=3
